simulink model "BLDC_Motor"  (R2018a)
settings: Solver=VariableStepAuto  StartTime=0.0  StopTime=50  RelTol=1e-3
model workspace (MAT data in the model file):
  B = 5.2e-05
  J = 0.0007
  Ke = 0.0071
  Kt = 0.0071
  L = 0.0005
  P = 4
  R = 3.25
libraries: simulink x10, simulink_extras x6
settings Model: Creator=Siddharth Deore  LastModifiedBy=Siddharth Deore

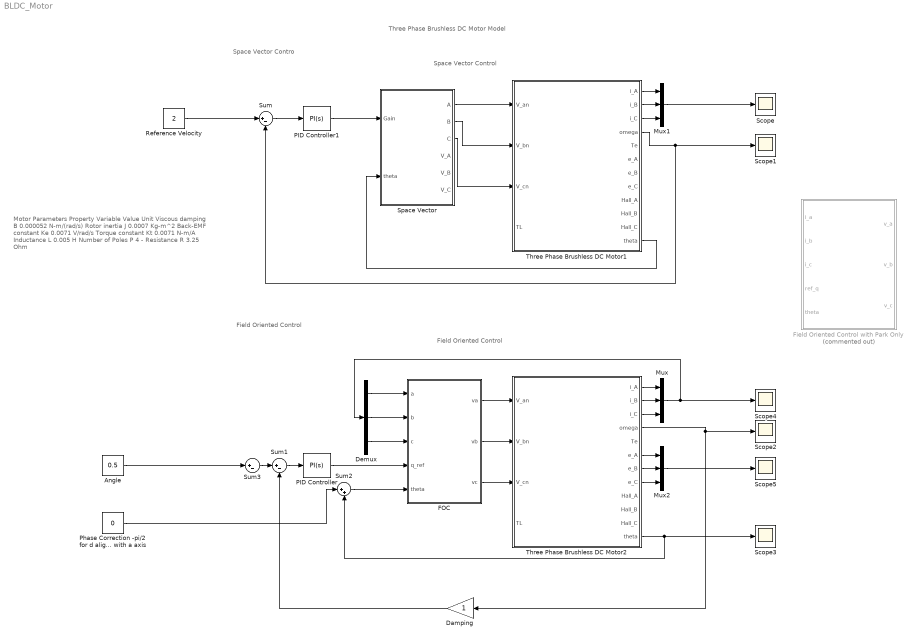
== system BLDC_Motor ==
  note: Motor Parameters
      |
      | Property
      | Variable
      | Value
      | Unit
      |
      | Viscous damping
      | B
      | 0.000052
      | N-m/(rad/s)
      |
      | Rotor inertia
      | J
      | 0.0007
      | Kg-m^2
      |
      | Back-EMF constant
      | Ke
      | 0.0071
      | V/rad/s
      |
      | Torque constant
      | Kt
      | 0.0071
      | N-m/A
      |
      | Inductance
      | L
      | 0.005
      | H
      |
      | Number of Poles
      | P
      | 4
      | -
      |
      | Resistance
      | R
      | 3.25
      | Ohm
  note: Field Oriented Control
  note: Space Vector Contro
  note: Space Vector Control
  note: Three Phase Brushless DC Motor Model
  note: Field Oriented Control
  Angle : Constant  Value=0.5
  Damping : Gain
  Demux : Demux  Outputs=3
  FOC : Subsystem
  Field Oriented Control with Park Only : Subsystem  Commented=on
  Mux : Mux  Inputs=3
  Mux1 : Mux  Inputs=3
  Mux2 : Mux  Inputs=3
  PID Controller : simulink/Continuous/PID Controller  Controller=PI  TimeDomain=Continuous-time  SampleTime=-1  IntegratorMethod=Forward Euler  FilterMethod=Forward Euler  Form=Parallel  UseFilter=on  ControllerParametersSource=internal  P=7  I=0.1  D=0.2  N=100  InitialConditionSource=internal  InitialConditionForIntegrator=0  InitialConditionForFilter=0  ExternalReset=none  LimitOutput=off  UpperSaturationLimit=inf  LowerSaturationLimit=-inf  LinearizeAsGain=on  AntiWindupMode=none  Kb=1  TrackingMode=off  Kt=1  PParamMin=[]  PParamMax=[]  IParamMin=[]  IParamMax=[]  DParamMin=[]  DParamMax=[]  NParamMin=[]  NParamMax=[]  KbParamMin=[]  KbParamMax=[]  KtParamMin=[]  KtParamMax=[]  POutMin=[]  POutMax=[]  IOutMin=[]  IOutMax=[]  DOutMin=[]  DOutMax=[]  NOutMin=[]  NOutMax=[]  KbOutMin=[]  KbOutMax=[]  KtOutMin=[]  KtOutMax=[]  IntegratorOutMin=[]  IntegratorOutMax=[]  FilterOutMin=[]  FilterOutMax=[]  SumOutMin=[]  SumOutMax=[]  SumI1OutMin=[]  SumI1OutMax=[]  SumI2OutMin=[]  SumI2OutMax=[]  SumI3OutMin=[]  SumI3OutMax=[]  SumDOutMin=[]  SumDOutMax=[]  SaturationOutMin=[]  SaturationOutMax=[]  IntegratorContinuousStateAttributes=''  IntegratorStateMustResolveToSignalObject=off  IntegratorRTWStateStorageClass=Auto  FilterContinuousStateAttributes=''  FilterStateMustResolveToSignalObject=off  FilterRTWStateStorageClass=Auto  DifferentiatorICPrevScaledInput=0  DifferentiatorOutMin=[]  DifferentiatorOutMax=[]  FilterDiffOutCoefMin=[]  FilterDiffOutCoefMax=[]  SumDenOutMin=[]  SumDenOutMax=[]  SumNumOutMin=[]  SumNumOutMax=[]  ReciprocalOutMin=[]  ReciprocalOutMax=[]  DivideOutMin=[]  DivideOutMax=[]  TunerSelectOption=Transfer Function Based (PID Tuner App)
  PID Controller1 : simulink/Continuous/PID Controller  Controller=PI  TimeDomain=Continuous-time  SampleTime=-1  IntegratorMethod=Forward Euler  FilterMethod=Forward Euler  Form=Parallel  UseFilter=on  ControllerParametersSource=internal  P=10  I=0.01  D=1  N=100  InitialConditionSource=internal  InitialConditionForIntegrator=0  InitialConditionForFilter=0  ExternalReset=none  LimitOutput=off  UpperSaturationLimit=inf  LowerSaturationLimit=-inf  LinearizeAsGain=on  AntiWindupMode=none  Kb=1  TrackingMode=off  Kt=1  PParamMin=[]  PParamMax=[]  IParamMin=[]  IParamMax=[]  DParamMin=[]  DParamMax=[]  NParamMin=[]  NParamMax=[]  KbParamMin=[]  KbParamMax=[]  KtParamMin=[]  KtParamMax=[]  POutMin=[]  POutMax=[]  IOutMin=[]  IOutMax=[]  DOutMin=[]  DOutMax=[]  NOutMin=[]  NOutMax=[]  KbOutMin=[]  KbOutMax=[]  KtOutMin=[]  KtOutMax=[]  IntegratorOutMin=[]  IntegratorOutMax=[]  FilterOutMin=[]  FilterOutMax=[]  SumOutMin=[]  SumOutMax=[]  SumI1OutMin=[]  SumI1OutMax=[]  SumI2OutMin=[]  SumI2OutMax=[]  SumI3OutMin=[]  SumI3OutMax=[]  SumDOutMin=[]  SumDOutMax=[]  SaturationOutMin=[]  SaturationOutMax=[]  IntegratorContinuousStateAttributes=''  IntegratorStateMustResolveToSignalObject=off  IntegratorRTWStateStorageClass=Auto  FilterContinuousStateAttributes=''  FilterStateMustResolveToSignalObject=off  FilterRTWStateStorageClass=Auto  DifferentiatorICPrevScaledInput=0  DifferentiatorOutMin=[]  DifferentiatorOutMax=[]  FilterDiffOutCoefMin=[]  FilterDiffOutCoefMax=[]  SumDenOutMin=[]  SumDenOutMax=[]  SumNumOutMin=[]  SumNumOutMax=[]  ReciprocalOutMin=[]  ReciprocalOutMax=[]  DivideOutMin=[]  DivideOutMax=[]  TunerSelectOption=Transfer Function Based (PID Tuner App)
  Phase Correction -pi/2 for d aligend with a axis : Constant  Value=0
  "Reference Velocity " : Constant  Value=2
  Scope{,1..5} (6 alike) : Scope
  Space Vector : Subsystem
  Sum : Sum  Inputs=|+-
  Sum1 : Sum  Inputs=|+-
  Sum2 : Sum  Inputs=|++
  Sum3 : Sum  Inputs=|+-
  Three Phase Brushless DC Motor1 : Subsystem  mask{B=0.000052, J=0.0007, Ke=0.0071, Kt=0.0071, L=0.005, P=4, R=3.25}
      mask prompts: B "Viscous damping [Nm/(rad/sec)]"; J "Innertia [Kg m^2]"; Ke "Back-EMF constant [V/rad/sec]"; Kt "Torque constant [Nm/A]"; L "Mutual Inductance [H]"; P "Number of Pole Pairs"; R "Coil Resistance [Ohm]"
  Three Phase Brushless DC Motor2 : Subsystem  mask{B=0.000052, J=0.0007, Ke=0.0071, Kt=0.0071, L=0.005, P=4, R=3.25}
      mask prompts: B "Viscous damping [Nm/(rad/sec)]"; J "Innertia [Kg m^2]"; Ke "Back-EMF constant [V/rad/sec]"; Kt "Torque constant [Nm/A]"; L "Mutual Inductance [H]"; P "Number of Pole Pairs"; R "Coil Resistance [Ohm]"
  wires:
  Sum/1 -> PID Controller1/1
  Space Vector/1(A) -> Three Phase Brushless DC Motor1/1(V_an)
  Space Vector/2(B) -> Three Phase Brushless DC Motor1/2(V_bn)
  Space Vector/3(C) -> Three Phase Brushless DC Motor1/3(V_cn)
  Three Phase Brushless DC Motor2/4(omega) -> Damping/1, Scope2/1
  Three Phase Brushless DC Motor2/12(theta) -> Sum2/2, Scope3/1
  Three Phase Brushless DC Motor2/1(i_A) -> Mux/1
  Three Phase Brushless DC Motor2/2(i_B) -> Mux/2
  Three Phase Brushless DC Motor2/3(i_C) -> Mux/3
  Mux/1 -> Scope4/1, Demux/1
  Demux/1 -> FOC/1(a)
  Demux/2 -> FOC/2(b)
  Demux/3 -> FOC/3(c)
  Sum1/1 -> PID Controller/1
  Three Phase Brushless DC Motor1/4(omega) -> Sum/2, Scope1/1
  Three Phase Brushless DC Motor1/12(theta) -> Space Vector/2(theta)
  PID Controller1/1 -> Space Vector/1(Gain)
  Angle/1 -> Sum3/1
  Sum3/1 -> Sum1/1
  "Reference Velocity "/1 -> Sum/1
  Damping/1 -> Sum1/2
  Three Phase Brushless DC Motor1/1(i_A) -> Mux1/1
  Three Phase Brushless DC Motor1/2(i_B) -> Mux1/2
  Three Phase Brushless DC Motor1/3(i_C) -> Mux1/3
  Mux1/1 -> Scope/1
  Three Phase Brushless DC Motor2/6(e_A) -> Mux2/1
  Three Phase Brushless DC Motor2/7(e_B) -> Mux2/2
  Three Phase Brushless DC Motor2/8(e_C) -> Mux2/3
  Mux2/1 -> Scope5/1
  Phase Correction -pi/2 for d aligend with a axis/1 -> Sum2/1
  FOC/1(va) -> Three Phase Brushless DC Motor2/1(V_an)
  FOC/2(vb) -> Three Phase Brushless DC Motor2/2(V_bn)
  FOC/3(vc) -> Three Phase Brushless DC Motor2/3(V_cn)
  PID Controller/1 -> FOC/4(q_ref)
  Sum2/1 -> FOC/5("theta ")

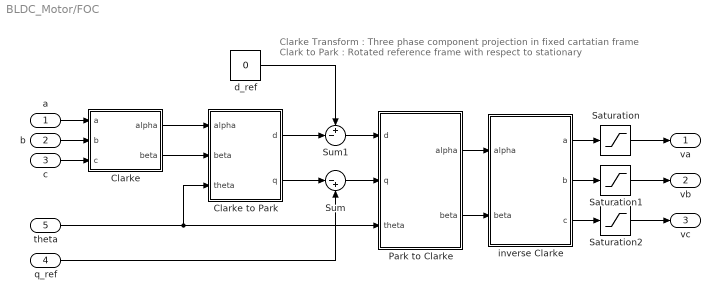
== system BLDC_Motor/FOC ==
  note: Clarke Transform : Three phase component projection in fixed cartatian frame
      | Clark to Park : Rotated reference frame with respect to stationary
  a : Inport
  b : Inport  Port=2
  c : Inport  Port=3
  q_ref : Inport  Port=4
  "theta " : Inport  Port=5
  Clarke : MATLAB Function  TreatAsAtomicUnit=on  VariantControl=Variant1
  Clarke to Park : MATLAB Function  TreatAsAtomicUnit=on
  Park to Clarke : MATLAB Function  TreatAsAtomicUnit=on
  Saturation : Saturate  UpperLimit=10  LowerLimit=-10
  Saturation1 : Saturate  UpperLimit=10  LowerLimit=-10
  Saturation2 : Saturate  UpperLimit=10  LowerLimit=-10
  Sum : Sum  Inputs=|-+
  Sum1 : Sum  Inputs=+-|
  d_ref : Constant  Value=0
  inverse Clarke : MATLAB Function  TreatAsAtomicUnit=on
  va : Outport
  vb : Outport  Port=2
  vc : Outport  Port=3
  wires:
  Clarke to Park/1(d) -> Sum1/2
  Clarke to Park/2(q) -> Sum/1
  "theta "/1 -> Clarke to Park/3(theta), Park to Clarke/3(theta)
  inverse Clarke/3(c) -> Saturation2/1
  inverse Clarke/1(a) -> Saturation/1
  q_ref/1 -> Sum/2
  Sum1/1 -> Park to Clarke/1(d)
  d_ref/1 -> Sum1/1
  inverse Clarke/2(b) -> Saturation1/1
  Park to Clarke/2(beta) -> inverse Clarke/2(beta)
  Park to Clarke/1(alpha) -> inverse Clarke/1(alpha)
  Sum/1 -> Park to Clarke/2(q)
  Saturation/1 -> va/1
  Saturation1/1 -> vb/1
  Saturation2/1 -> vc/1
  a/1 -> Clarke/1(a)
  b/1 -> Clarke/2(b)
  c/1 -> Clarke/3(c)
  Clarke/1(alpha) -> Clarke to Park/1(alpha)
  Clarke/2(beta) -> Clarke to Park/2(beta)

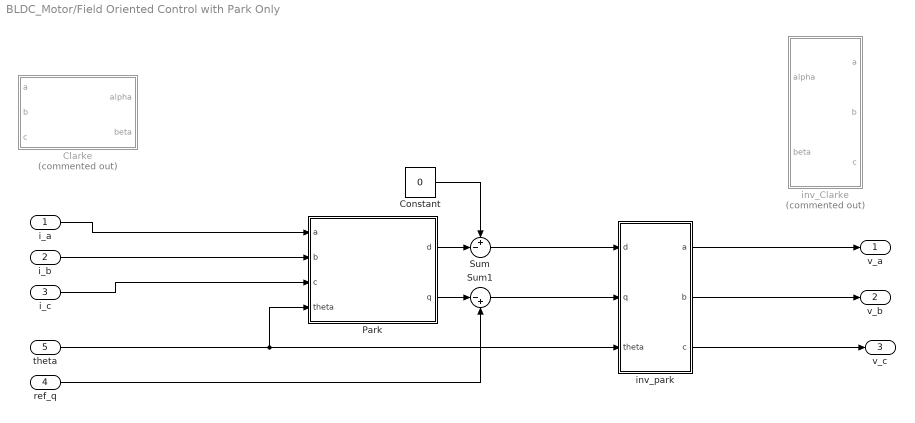
== system BLDC_Motor/Field Oriented Control with Park Only ==
  i_a : Inport
  i_b : Inport  Port=2
  i_c : Inport  Port=3
  ref_q : Inport  Port=4
  theta : Inport  Port=5
  Clarke : MATLAB Function  Commented=on  TreatAsAtomicUnit=on
  Constant : Constant  Value=0
  Park : MATLAB Function  TreatAsAtomicUnit=on
  Sum : Sum  Inputs=+-|
  Sum1 : Sum  Inputs=|-+
  inv_Clarke : MATLAB Function  Commented=on  TreatAsAtomicUnit=on
  inv_park : MATLAB Function  TreatAsAtomicUnit=on
  v_a : Outport
  v_b : Outport  Port=2
  v_c : Outport  Port=3
  wires:
  i_a/1 -> Park/1(a)
  i_b/1 -> Park/2(b)
  i_c/1 -> Park/3(c)
  theta/1 -> Park/4(theta), inv_park/3(theta)
  Sum/1 -> inv_park/1(d)
  Sum1/1 -> inv_park/2(q)
  Park/2(q) -> Sum1/1
  ref_q/1 -> Sum1/2
  Park/1(d) -> Sum/2
  Constant/1 -> Sum/1
  inv_park/1(a) -> v_a/1
  inv_park/2(b) -> v_b/1
  inv_park/3(c) -> v_c/1

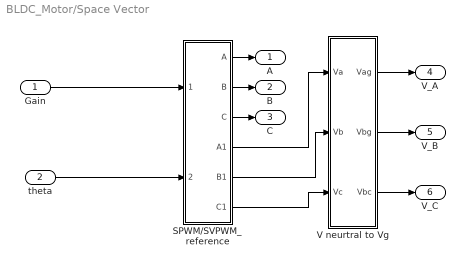
== system BLDC_Motor/Space Vector ==
  Gain : Inport
  theta : Inport  Port=2
  SPWM/SVPWM_reference : Subsystem
  V neurtral to Vg : Subsystem
  A : Outport
  B : Outport  Port=2
  C : Outport  Port=3
  V_A : Outport  Port=4
  V_B : Outport  Port=5
  V_C : Outport  Port=6
  wires:
  SPWM/SVPWM_reference/4(A1) -> V neurtral to Vg/1(Va)
  V neurtral to Vg/1(Vag) -> V_A/1
  SPWM/SVPWM_reference/6(C1) -> V neurtral to Vg/3(Vc)
  SPWM/SVPWM_reference/2(B) -> B/1
  SPWM/SVPWM_reference/5(B1) -> V neurtral to Vg/2(Vb)
  theta/1 -> SPWM/SVPWM_reference/2(theta)
  Gain/1 -> SPWM/SVPWM_reference/1(Gain)
  V neurtral to Vg/3(Vbc) -> V_C/1
  SPWM/SVPWM_reference/1(A) -> A/1
  V neurtral to Vg/2(Vbg) -> V_B/1
  SPWM/SVPWM_reference/3(C) -> C/1

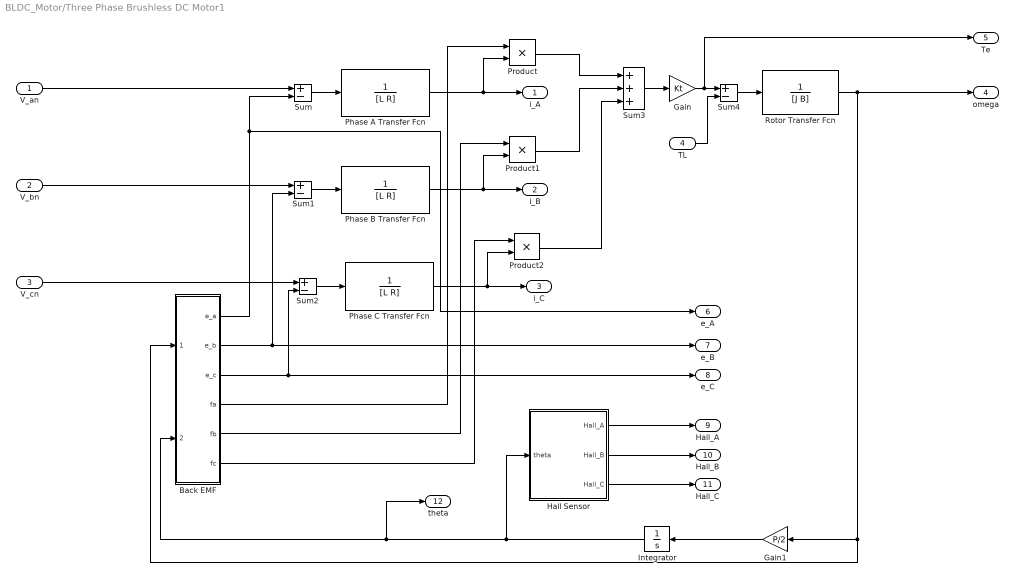
== system BLDC_Motor/Three Phase Brushless DC Motor1 ==
  V_an : Inport
  V_bn : Inport  Port=2
  V_cn : Inport  Port=3
  TL : Inport  Port=4
  Back EMF : Subsystem
  Gain : Gain  Gain=Kt
  Gain1 : Gain  Gain=P/2
  Hall Sensor : Subsystem
  Integrator : Integrator
  Phase A Transfer Fcn : TransferFcn  Denominator=[L R]
  Phase B Transfer Fcn : TransferFcn  Denominator=[L R]
  Phase C Transfer Fcn : TransferFcn  Denominator=[L R]
  Product : Product
  Product1 : Product
  Product2 : Product
  Rotor Transfer Fcn : TransferFcn  Denominator=[J B]
  Sum{,1..2,4} (4 alike) : Sum  Inputs=+-
  Sum3 : Sum  Inputs=+++
  i_A : Outport
  i_B : Outport  Port=2
  i_C : Outport  Port=3
  omega : Outport  Port=4
  Te : Outport  Port=5
  e_A : Outport  Port=6
  e_B : Outport  Port=7
  e_C : Outport  Port=8
  Hall_A : Outport  Port=9
  Hall_B : Outport  Port=10
  Hall_C : Outport  Port=11
  theta : Outport  Port=12
  wires:
  Integrator/1 -> theta/1, Back EMF/2(theta), Hall Sensor/1(theta)
  Back EMF/2(e_b) -> e_B/1, Sum1/2
  V_bn/1 -> Sum1/1
  Gain1/1 -> Integrator/1
  Product2/1 -> Sum3/3
  Rotor Transfer Fcn/1 -> omega/1, Back EMF/1(omega), Gain1/1
  Hall Sensor/2(Hall_B) -> Hall_B/1
  V_an/1 -> Sum/1
  Back EMF/6(fc) -> Product2/1
  Back EMF/3(e_c) -> e_C/1, Sum2/2
  Hall Sensor/3(Hall_C) -> Hall_C/1
  Back EMF/1(e_a) -> e_A/1, Sum/2
  Back EMF/5(fb) -> Product1/1
  Gain/1 -> Te/1, Sum4/1
  Sum2/1 -> Phase C Transfer Fcn/1
  Phase A Transfer Fcn/1 -> i_A/1, Product/2
  Back EMF/4(fa) -> Product/1
  Sum/1 -> Phase A Transfer Fcn/1
  Sum1/1 -> Phase B Transfer Fcn/1
  Phase C Transfer Fcn/1 -> i_C/1, Product2/2
  Product/1 -> Sum3/1
  Phase B Transfer Fcn/1 -> i_B/1, Product1/2
  Sum3/1 -> Gain/1
  V_cn/1 -> Sum2/1
  Product1/1 -> Sum3/2
  Hall Sensor/1(Hall_A) -> Hall_A/1
  TL/1 -> Sum4/2
  Sum4/1 -> Rotor Transfer Fcn/1

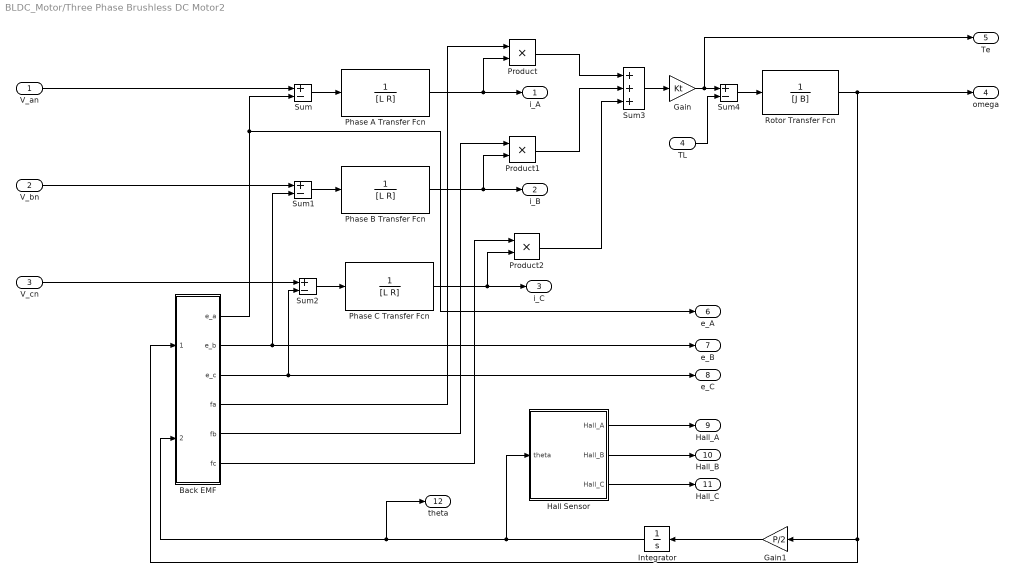
== system BLDC_Motor/Three Phase Brushless DC Motor2 ==
  V_an : Inport
  V_bn : Inport  Port=2
  V_cn : Inport  Port=3
  TL : Inport  Port=4
  Back EMF : Subsystem
  Gain : Gain  Gain=Kt
  Gain1 : Gain  Gain=P/2
  Hall Sensor : Subsystem
  Integrator : Integrator
  Phase A Transfer Fcn : TransferFcn  Denominator=[L R]
  Phase B Transfer Fcn : TransferFcn  Denominator=[L R]
  Phase C Transfer Fcn : TransferFcn  Denominator=[L R]
  Product : Product
  Product1 : Product
  Product2 : Product
  Rotor Transfer Fcn : TransferFcn  Denominator=[J B]
  Sum{,1..2,4} (4 alike) : Sum  Inputs=+-
  Sum3 : Sum  Inputs=+++
  i_A : Outport
  i_B : Outport  Port=2
  i_C : Outport  Port=3
  omega : Outport  Port=4
  Te : Outport  Port=5
  e_A : Outport  Port=6
  e_B : Outport  Port=7
  e_C : Outport  Port=8
  Hall_A : Outport  Port=9
  Hall_B : Outport  Port=10
  Hall_C : Outport  Port=11
  theta : Outport  Port=12
  wires:
  Integrator/1 -> theta/1, Back EMF/2(theta), Hall Sensor/1(theta)
  Back EMF/2(e_b) -> e_B/1, Sum1/2
  V_bn/1 -> Sum1/1
  Gain1/1 -> Integrator/1
  Product2/1 -> Sum3/3
  Rotor Transfer Fcn/1 -> omega/1, Back EMF/1(omega), Gain1/1
  Hall Sensor/2(Hall_B) -> Hall_B/1
  V_an/1 -> Sum/1
  Back EMF/6(fc) -> Product2/1
  Back EMF/3(e_c) -> e_C/1, Sum2/2
  Hall Sensor/3(Hall_C) -> Hall_C/1
  Back EMF/1(e_a) -> e_A/1, Sum/2
  Back EMF/5(fb) -> Product1/1
  Gain/1 -> Te/1, Sum4/1
  Sum2/1 -> Phase C Transfer Fcn/1
  Phase A Transfer Fcn/1 -> i_A/1, Product/2
  Back EMF/4(fa) -> Product/1
  Sum/1 -> Phase A Transfer Fcn/1
  Sum1/1 -> Phase B Transfer Fcn/1
  Phase C Transfer Fcn/1 -> i_C/1, Product2/2
  Product/1 -> Sum3/1
  Phase B Transfer Fcn/1 -> i_B/1, Product1/2
  Sum3/1 -> Gain/1
  V_cn/1 -> Sum2/1
  Product1/1 -> Sum3/2
  Hall Sensor/1(Hall_A) -> Hall_A/1
  TL/1 -> Sum4/2
  Sum4/1 -> Rotor Transfer Fcn/1

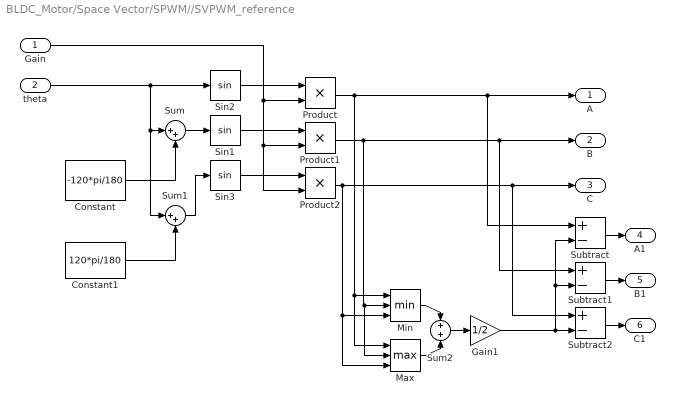
== system BLDC_Motor/Space Vector/SPWM//SVPWM_reference ==
  Gain : Inport
  theta : Inport  Port=2
  Constant : Constant  Value=-120*pi/180
  Constant1 : Constant  Value=120*pi/180
  Gain1 : Gain  Gain=1/2
  Max : MinMax  Function=max  Inputs=3
  Min : MinMax  Inputs=3
  Product : Product
  Product1 : Product
  Product2 : Product
  Sin1 : Trigonometry
  Sin2 : Trigonometry
  Sin3 : Trigonometry
  Subtract : Sum  Inputs=+-
  Subtract1 : Sum  Inputs=+-
  Subtract2 : Sum  Inputs=+-
  Sum : Sum  Inputs=|++
  Sum1 : Sum  Inputs=|++
  Sum2 : Sum
  A : Outport
  B : Outport  Port=2
  C : Outport  Port=3
  A1 : Outport  Port=4
  B1 : Outport  Port=5
  C1 : Outport  Port=6
  wires:
  Product/1 -> Min/1, Max/1, Subtract/1, A/1
  Product1/1 -> Max/2, Min/2, Subtract1/1, B/1
  Product2/1 -> Max/3, Min/3, Subtract2/1, C/1
  Sin2/1 -> Product/1
  Gain/1 -> Product2/2, Product1/2, Product/2
  Sin1/1 -> Product1/1
  Sum/1 -> Sin1/1
  Constant/1 -> Sum/2
  Sum1/1 -> Sin3/1
  Sin3/1 -> Product2/1
  Constant1/1 -> Sum1/2
  theta/1 -> Sum1/1, Sum/1, Sin2/1
  Min/1 -> Sum2/1
  Max/1 -> Sum2/2
  Sum2/1 -> Gain1/1
  Subtract/1 -> A1/1
  Subtract1/1 -> B1/1
  Gain1/1 -> Subtract/2, Subtract1/2, Subtract2/2
  Subtract2/1 -> C1/1

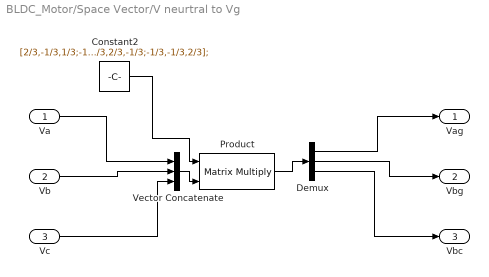
== system BLDC_Motor/Space Vector/V neurtral to Vg ==
  Va : Inport
  Vb : Inport  Port=2
  Vc : Inport  Port=3
  Constant2 : Constant  Value=[2/3,-1/3,1/3;-1/3,2/3,-1/3;-1/3,-1/3,2/3];
  Demux : Demux  Outputs=3
  Product : Product  Multiplication=Matrix(*)
  Vector Concatenate : Concatenate  NumInputs=3
  Vag : Outport
  Vbg : Outport  Port=2
  Vbc : Outport  Port=3
  wires:
  Vb/1 -> Vector Concatenate/2
  Demux/2 -> Vbg/1
  Demux/3 -> Vbc/1
  Vc/1 -> Vector Concatenate/3
  Vector Concatenate/1 -> Product/2
  Product/1 -> Demux/1
  Va/1 -> Vector Concatenate/1
  Constant2/1 -> Product/1
  Demux/1 -> Vag/1

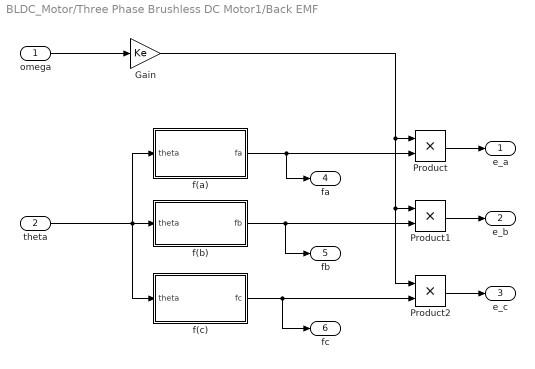
== system BLDC_Motor/Three Phase Brushless DC Motor1/Back EMF ==
  omega : Inport
  theta : Inport  Port=2
  Gain : Gain  Gain=Ke
  Product : Product
  Product1 : Product
  Product2 : Product
  f(a) : Subsystem
  f(b) : Subsystem
  f(c) : Subsystem
  e_a : Outport
  e_b : Outport  Port=2
  e_c : Outport  Port=3
  fa : Outport  Port=4
  fb : Outport  Port=5
  fc : Outport  Port=6
  wires:
  omega/1 -> Gain/1
  Product/1 -> e_a/1
  Product1/1 -> e_b/1
  Product2/1 -> e_c/1
  Gain/1 -> Product2/1, Product1/1, Product/1
  f(a)/1(fa) -> fa/1, Product/2
  f(b)/1(fb) -> fb/1, Product1/2
  f(c)/1(fc) -> fc/1, Product2/2
  theta/1 -> f(c)/1(theta), f(a)/1(theta), f(b)/1(theta)

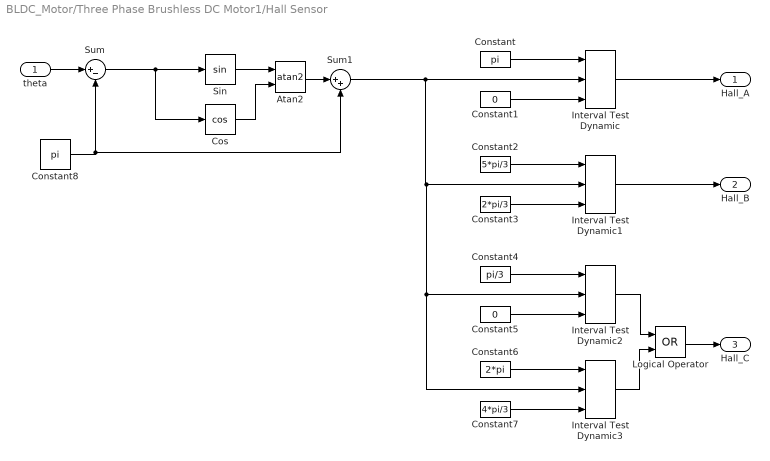
== system BLDC_Motor/Three Phase Brushless DC Motor1/Hall Sensor ==
  theta : Inport
  Atan2 : Trigonometry  Operator=atan2
  Constant : Constant  Value=pi
  Constant1 : Constant  Value=0
  Constant2 : Constant  Value=5*pi/3
  Constant3 : Constant  Value=2*pi/3
  Constant4 : Constant  Value=pi/3
  Constant5 : Constant  Value=0
  Constant6 : Constant  Value=2*pi
  Constant7 : Constant  Value=4*pi/3
  Constant8 : Constant  Value=pi
  Cos : Trigonometry  Operator=cos
  Interval Test Dynamic{,1..3} (4 alike) : simulink/Logic and Bit Operations/Interval Test Dynamic  IntervalClosedRight=on  IntervalClosedLeft=on  OutDataTypeStr=boolean
      settings: SourceProductName=Simulink  SourceProductBaseCode=SL
  Logical Operator : Logic  Operator=OR  AllPortsSameDT=off  OutDataTypeStr=boolean
  Sin : Trigonometry
  Sum : Sum  Inputs=|+-
  Sum1 : Sum  Inputs=|++
  Hall_A : Outport
  Hall_B : Outport  Port=2
  Hall_C : Outport  Port=3
  wires:
  Constant/1 -> Interval Test Dynamic/1
  Constant1/1 -> Interval Test Dynamic/3
  Constant3/1 -> Interval Test Dynamic1/3
  Constant2/1 -> Interval Test Dynamic1/1
  Constant5/1 -> Interval Test Dynamic2/3
  Constant4/1 -> Interval Test Dynamic2/1
  Constant7/1 -> Interval Test Dynamic3/3
  Constant6/1 -> Interval Test Dynamic3/1
  Interval Test Dynamic2/1 -> Logical Operator/1
  Interval Test Dynamic3/1 -> Logical Operator/2
  Logical Operator/1 -> Hall_C/1
  Interval Test Dynamic1/1 -> Hall_B/1
  Interval Test Dynamic/1 -> Hall_A/1
  Sin/1 -> Atan2/1
  Cos/1 -> Atan2/2
  theta/1 -> Sum/1
  Atan2/1 -> Sum1/1
  Sum/1 -> Cos/1, Sin/1
  Constant8/1 -> Sum1/2, Sum/2
  Sum1/1 -> Interval Test Dynamic3/2, Interval Test Dynamic2/2, Interval Test Dynamic1/2, Interval Test Dynamic/2

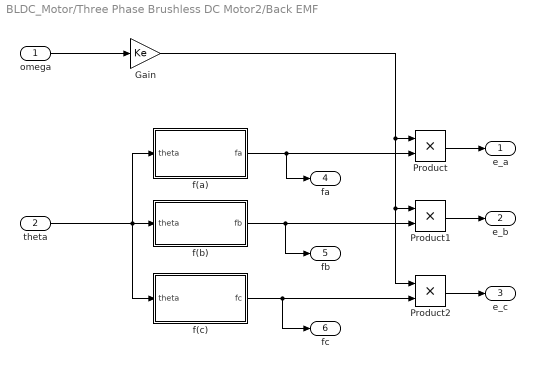
== system BLDC_Motor/Three Phase Brushless DC Motor2/Back EMF ==
  omega : Inport
  theta : Inport  Port=2
  Gain : Gain  Gain=Ke
  Product : Product
  Product1 : Product
  Product2 : Product
  f(a) : Subsystem
  f(b) : Subsystem
  f(c) : Subsystem
  e_a : Outport
  e_b : Outport  Port=2
  e_c : Outport  Port=3
  fa : Outport  Port=4
  fb : Outport  Port=5
  fc : Outport  Port=6
  wires:
  omega/1 -> Gain/1
  Product/1 -> e_a/1
  Product1/1 -> e_b/1
  Product2/1 -> e_c/1
  Gain/1 -> Product2/1, Product1/1, Product/1
  f(a)/1(fa) -> fa/1, Product/2
  f(b)/1(fb) -> fb/1, Product1/2
  f(c)/1(fc) -> fc/1, Product2/2
  theta/1 -> f(c)/1(theta), f(a)/1(theta), f(b)/1(theta)

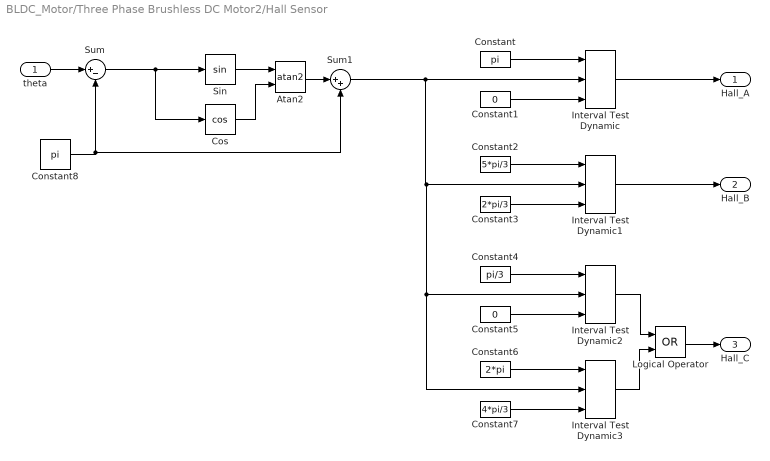
== system BLDC_Motor/Three Phase Brushless DC Motor2/Hall Sensor ==
  theta : Inport
  Atan2 : Trigonometry  Operator=atan2
  Constant : Constant  Value=pi
  Constant1 : Constant  Value=0
  Constant2 : Constant  Value=5*pi/3
  Constant3 : Constant  Value=2*pi/3
  Constant4 : Constant  Value=pi/3
  Constant5 : Constant  Value=0
  Constant6 : Constant  Value=2*pi
  Constant7 : Constant  Value=4*pi/3
  Constant8 : Constant  Value=pi
  Cos : Trigonometry  Operator=cos
  Interval Test Dynamic{,1..3} (4 alike) : simulink/Logic and Bit Operations/Interval Test Dynamic  IntervalClosedRight=on  IntervalClosedLeft=on  OutDataTypeStr=boolean
      settings: SourceProductName=Simulink  SourceProductBaseCode=SL
  Logical Operator : Logic  Operator=OR  AllPortsSameDT=off  OutDataTypeStr=boolean
  Sin : Trigonometry
  Sum : Sum  Inputs=|+-
  Sum1 : Sum  Inputs=|++
  Hall_A : Outport
  Hall_B : Outport  Port=2
  Hall_C : Outport  Port=3
  wires:
  Constant/1 -> Interval Test Dynamic/1
  Constant1/1 -> Interval Test Dynamic/3
  Constant3/1 -> Interval Test Dynamic1/3
  Constant2/1 -> Interval Test Dynamic1/1
  Constant5/1 -> Interval Test Dynamic2/3
  Constant4/1 -> Interval Test Dynamic2/1
  Constant7/1 -> Interval Test Dynamic3/3
  Constant6/1 -> Interval Test Dynamic3/1
  Interval Test Dynamic2/1 -> Logical Operator/1
  Interval Test Dynamic3/1 -> Logical Operator/2
  Logical Operator/1 -> Hall_C/1
  Interval Test Dynamic1/1 -> Hall_B/1
  Interval Test Dynamic/1 -> Hall_A/1
  Sin/1 -> Atan2/1
  Cos/1 -> Atan2/2
  theta/1 -> Sum/1
  Atan2/1 -> Sum1/1
  Sum/1 -> Cos/1, Sin/1
  Constant8/1 -> Sum1/2, Sum/2
  Sum1/1 -> Interval Test Dynamic3/2, Interval Test Dynamic2/2, Interval Test Dynamic1/2, Interval Test Dynamic/2

== system BLDC_Motor/Three Phase Brushless DC Motor1/Back EMF/f(a) ==
  theta : Inport
  Atan2 : Trigonometry  Operator=atan2
  Cos : Trigonometry  Operator=cos
  Radians to Degrees : simulink_extras/Transformations/Radians to Degrees
  Sin : Trigonometry
  Trapizoidal Lookup with Linear Point-slope Interpolation : Lookup_n-D  NumberOfTableDimensions=1  BreakpointsForDimension1="[-180,  -120,   -60,     0,    60,   120,   180]"  Table=[-1,-1,-1,1,1,1,-1]  InternalRulePriority=Speed  RndMeth=Simplest  InputSameDT=on
  fa : Outport
  wires:
  Trapizoidal Lookup with Linear Point-slope Interpolation/1 -> fa/1
  Cos/1 -> Atan2/2
  Sin/1 -> Atan2/1
  Radians to Degrees/1 -> Trapizoidal Lookup with Linear Point-slope Interpolation/1
  Atan2/1 -> Radians to Degrees/1
  theta/1 -> Cos/1, Sin/1

== system BLDC_Motor/Three Phase Brushless DC Motor1/Back EMF/f(b) ==
  theta : Inport
  Atan2 : Trigonometry  Operator=atan2
  Cos : Trigonometry  Operator=cos
  Radians to Degrees : simulink_extras/Transformations/Radians to Degrees
  Sin : Trigonometry
  Trapizoidal Lookup with Linear Point-slope Interpolation : Lookup_n-D  NumberOfTableDimensions=1  BreakpointsForDimension1="[-180,  -120,   -60,     0,    60,   120,   180]"  Table=[1,1,-1,-1,-1,1,1]  InternalRulePriority=Speed  RndMeth=Simplest  InputSameDT=on
  fb : Outport
  wires:
  Trapizoidal Lookup with Linear Point-slope Interpolation/1 -> fb/1
  Cos/1 -> Atan2/2
  Sin/1 -> Atan2/1
  Radians to Degrees/1 -> Trapizoidal Lookup with Linear Point-slope Interpolation/1
  Atan2/1 -> Radians to Degrees/1
  theta/1 -> Cos/1, Sin/1

== system BLDC_Motor/Three Phase Brushless DC Motor1/Back EMF/f(c) ==
  theta : Inport
  Atan2 : Trigonometry  Operator=atan2
  Cos : Trigonometry  Operator=cos
  Radians to Degrees : simulink_extras/Transformations/Radians to Degrees
  Sin : Trigonometry
  Trapizoidal Lookup with Linear Point-slope Interpolation : Lookup_n-D  NumberOfTableDimensions=1  BreakpointsForDimension1="[-180,  -120,   -60,     0,    60,   120,   180]"  Table=[-1,1,1,1,-1,-1,-1]  InternalRulePriority=Speed  RndMeth=Simplest  InputSameDT=on
  fc : Outport
  wires:
  Trapizoidal Lookup with Linear Point-slope Interpolation/1 -> fc/1
  Cos/1 -> Atan2/2
  Sin/1 -> Atan2/1
  Radians to Degrees/1 -> Trapizoidal Lookup with Linear Point-slope Interpolation/1
  Atan2/1 -> Radians to Degrees/1
  theta/1 -> Cos/1, Sin/1

== system BLDC_Motor/Three Phase Brushless DC Motor2/Back EMF/f(a) ==
  theta : Inport
  Atan2 : Trigonometry  Operator=atan2
  Cos : Trigonometry  Operator=cos
  Radians to Degrees : simulink_extras/Transformations/Radians to Degrees
  Sin : Trigonometry
  Trapizoidal Lookup with Linear Point-slope Interpolation : Lookup_n-D  NumberOfTableDimensions=1  BreakpointsForDimension1="[-180,  -120,   -60,     0,    60,   120,   180]"  Table=[-1,-1,-1,1,1,1,-1]  InternalRulePriority=Speed  RndMeth=Simplest  InputSameDT=on
  fa : Outport
  wires:
  Trapizoidal Lookup with Linear Point-slope Interpolation/1 -> fa/1
  Cos/1 -> Atan2/2
  Sin/1 -> Atan2/1
  Radians to Degrees/1 -> Trapizoidal Lookup with Linear Point-slope Interpolation/1
  Atan2/1 -> Radians to Degrees/1
  theta/1 -> Cos/1, Sin/1

== system BLDC_Motor/Three Phase Brushless DC Motor2/Back EMF/f(b) ==
  theta : Inport
  Atan2 : Trigonometry  Operator=atan2
  Cos : Trigonometry  Operator=cos
  Radians to Degrees : simulink_extras/Transformations/Radians to Degrees
  Sin : Trigonometry
  Trapizoidal Lookup with Linear Point-slope Interpolation : Lookup_n-D  NumberOfTableDimensions=1  BreakpointsForDimension1="[-180,  -120,   -60,     0,    60,   120,   180]"  Table=[1,1,-1,-1,-1,1,1]  InternalRulePriority=Speed  RndMeth=Simplest  InputSameDT=on
  fb : Outport
  wires:
  Trapizoidal Lookup with Linear Point-slope Interpolation/1 -> fb/1
  Cos/1 -> Atan2/2
  Sin/1 -> Atan2/1
  Radians to Degrees/1 -> Trapizoidal Lookup with Linear Point-slope Interpolation/1
  Atan2/1 -> Radians to Degrees/1
  theta/1 -> Cos/1, Sin/1

== system BLDC_Motor/Three Phase Brushless DC Motor2/Back EMF/f(c) ==
  theta : Inport
  Atan2 : Trigonometry  Operator=atan2
  Cos : Trigonometry  Operator=cos
  Radians to Degrees : simulink_extras/Transformations/Radians to Degrees
  Sin : Trigonometry
  Trapizoidal Lookup with Linear Point-slope Interpolation : Lookup_n-D  NumberOfTableDimensions=1  BreakpointsForDimension1="[-180,  -120,   -60,     0,    60,   120,   180]"  Table=[-1,1,1,1,-1,-1,-1]  InternalRulePriority=Speed  RndMeth=Simplest  InputSameDT=on
  fc : Outport
  wires:
  Trapizoidal Lookup with Linear Point-slope Interpolation/1 -> fc/1
  Cos/1 -> Atan2/2
  Sin/1 -> Atan2/1
  Radians to Degrees/1 -> Trapizoidal Lookup with Linear Point-slope Interpolation/1
  Atan2/1 -> Radians to Degrees/1
  theta/1 -> Cos/1, Sin/1

== matlab function BLDC_Motor/Field Oriented Control with Park Only/inv_Clarke ==
  data: alpha input; a output; beta input; b output; c output
function [a,b,c]= fcn(alpha,beta)
% alpha-beta to  abc
%
a = alpha;
b = -0.5*alpha+0.8660*beta;
c = -0.5*alpha-0.8660*beta;

== matlab function BLDC_Motor/Field Oriented Control with Park Only/Clarke ==
  data: a input; alpha output; b input; c input; beta output
function [alpha,beta]= fcn(a,b,c)
% abc to alpha beta
% Clarke Transform
%T = [
 %   0.6667   -0.3333   -0.3333;
 %        0    1.1547   -1.1547;
 %        ];
%u=T*[a;b;c];
alpha = a;%;u(1);
beta =  0.5774*(a+2*b);%;u(2);

== matlab function BLDC_Motor/Field Oriented Control with Park Only/Park ==
  data: a input; d output; b input; c input; theta input; q output
function [d,q]= fcn(a,b,c,theta)
% Original Park Transform
% abc to dq,  a align to q
%T = 0.8165*[
%    sin(theta), sin(theta-2*pi/3), sin(theta+2*pi/3);
%    cos(theta), cos(theta-2*pi/3), cos(theta+2*pi/3);
%    0.7071,0.7071,0.7071];

% abc to dq,  a align to d

T = 2/3*[
    cos(theta), cos(theta-2*pi/3), cos(theta+2*pi/3);
    -sin(theta), -sin(theta-2*pi/3), -sin(theta+2*pi/3);
    0.5,0.5,0.5];
y=T*[a;b;c];
d = y(1);
q = y(2);

% Simple but inverse not working
%d = alpha * cos(theta) + beta * sin(theta);
%q = beta * cos(theta) - alpha * sin(theta);

== matlab function BLDC_Motor/Field Oriented Control with Park Only/inv_park ==
  data: d input; a output; q input; b output; theta input; c output
function [a,b,c]= fcn(d,q,theta)
% dq to abc, a aligned to q
%T=0.8165*[
%    sin(theta),        cos(theta),            0.7071;
%    sin(theta-2*pi/3), cos(theta-2*pi/3),     0.7071;
%    sin(theta+2*pi/3), cos(theta+2*pi/3),     0.7071];

% dq to abc, a aligned to d
T=[
    cos(theta),         -sin(theta),          1;
    cos(theta-2*pi/3), -sin(theta-2*pi/3),    1;
    cos(theta+2*pi/3), -sin(theta+2*pi/3),    1];
y=T*[d;q;0];
a = y(1);
b = y(2);
c = y(3);
% Simple but inverse not working
%alpha = d * cos(theta) - q * sin(theta)
%beta = q * cos(theta) + d * sin(theta)

== matlab function BLDC_Motor/FOC/Clarke ==
  data: a input; alpha output; b input; c input; beta output
function [alpha,beta] = fcn(a,b,c)
% Clarke Transform
T=2/3*[ 1,   -0.5,    -0.5;
        0, 0.8660, -0.8660;
        0.5,  0.5,    0.5];
y=T*[a;b;c];
alpha = y(1);
beta = y(2);

% sqrt(3)/2 = 0.8660

== matlab function BLDC_Motor/FOC/Clarke to Park ==
  data: alpha input; d output; beta input; theta input; q output
function [d,q] = fcn(alpha,beta,theta)
% d axis
%T=[cos(theta), sin(theta),0;
%-sin(theta),cos(theta),0
%0,0,1];
% q axis
 T=[sin(theta),-cos(theta),0;
 cos(theta),sin(theta),0
 0,0,1];

y=T*[alpha;beta;0];
d=y(1);
q=y(2);

== matlab function BLDC_Motor/FOC/Park to Clarke ==
  data: d input; alpha output; q input; theta input; beta output
function [alpha,beta] = fcn(d,q,theta)
% d axis
% T=[cos(theta), -sin(theta),0;
% sin(theta),cos(theta),0
% 0,0,1];
% q axis
 T=[sin(theta),cos(theta),0;
 -cos(theta),sin(theta),0
 0,0,1];
y=T*[d;q;0];
alpha = y(1);
beta = y(2);

== matlab function BLDC_Motor/FOC/inverse Clarke ==
  data: alpha input; a output; beta input; b output; c output
function [a,b,c] = fcn(alpha,beta)
% inverse Clarke
T=[    1.0000         0    1.0000;
   -0.5000    0.8661    1.0000;
   -0.5000   -0.8661    1.0000;];
y=T*[alpha;beta;0];
a=y(1);
b=y(2);
c=y(3);
